simulink model "Inverterfullbridge_rl_load"  (R2023b)
settings: Solver=VariableStepAuto  StartTime=0.0  StopTime=1  RelTol=1e-3
libraries: spsIGBTDiodeLib x4, spsVoltageMeasurementLib x2, spsCurrentMeasurementLib x1, spsDCVoltageSourceLib x1, spsSeriesRLCBranchLib x1, sps_lib x1
settings Model: Creator=junio  LastModifiedBy=Anuj

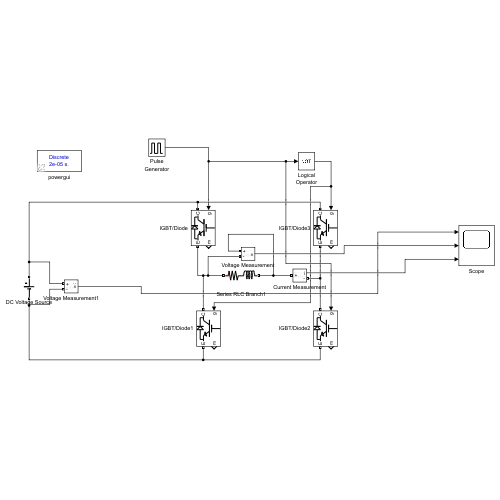
[thumbnail: Simulink's stored preview of the top-level diagram]
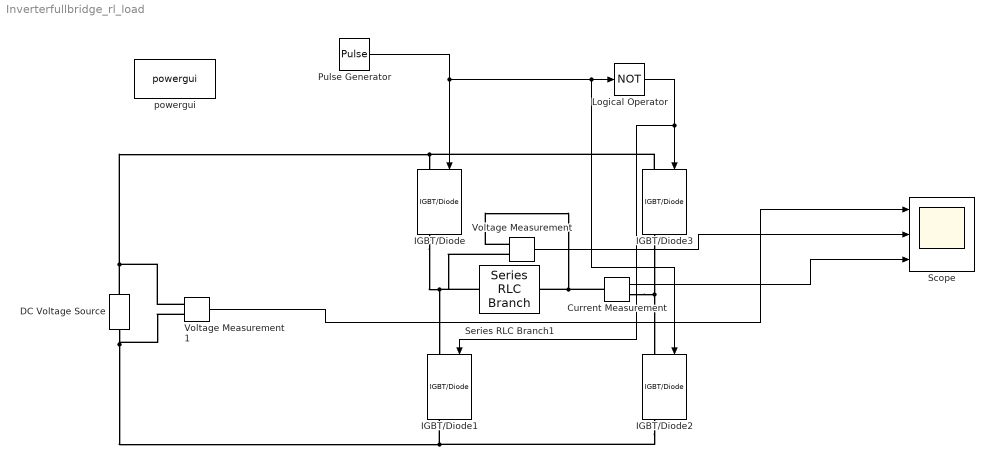
== system Inverterfullbridge_rl_load ==
  Current Measurement : spsCurrentMeasurementLib/Current Measurement  PhasorSimulation=off  OutputType=Complex  PSBequivalent=0
  DC Voltage Source : spsDCVoltageSourceLib/DC Voltage Source  Amplitude=24  Measurements=None
  IGBT/Diode{,1..3} (4 alike) : spsIGBTDiodeLib/IGBT//Diode  Ron=1e-3  Rs=1e5  Cs=inf  Measurements=on
  Logical Operator : Logic  Operator=NOT  AllPortsSameDT=off  OutDataTypeStr=boolean
  Pulse Generator : DiscretePulseGenerator  PulseType=Time based  Period=1/50  PulseWidth=50
  Scope : Scope  NumInputPorts=3
  Series RLC Branch1 : spsSeriesRLCBranchLib/Series RLC Branch  LConnTagsString=__new0  RConnTagsString=__new0  BranchType=RL  Resistance=10  Inductance=5e-3  SetiL0=off  InitialCurrent=0  Capacitance=1e-6  Setx0=off  InitialVoltage=0  Measurements=None
  Voltage Measurement : spsVoltageMeasurementLib/Voltage Measurement  PhasorSimulation=off  OutputType=Complex  PSBequivalent=0
  Voltage Measurement1 : spsVoltageMeasurementLib/Voltage Measurement  PhasorSimulation=off  OutputType=Complex  PSBequivalent=0
  powergui : sps_lib/powergui  Priority=1  SimulationMode=Discrete  SampleTime=2e-05  frequency=60  Iterations=50  frequencyindice=0  Pbase=100e6  ErrMax=1e-4  UnitsV=kV  UnitsW=MW  buscounter=0  FunctionMessages=off  echomessages=off  EnableUseOfTLC=off  CurrentSourceSwitches=off  DisableSnubberDevices=off  DisableRonSwitches=off  DisableVfSwitches=off  DisplayEquations=off  AutomaticDiscreteSolvers=off  SolverType=Tustin/Backward Euler (TBE)  Interpol=off  ExternalGateDelay=off  methode=off  Ts=100  x0status=blocks  SPID=on  SwTol=0  HookPort=off  NonlinearTolerance=1e-4  nMaxIteration=100  ContinueOnMaxIteration=off  RestoreLinks=warning  ResistiveCurrentMeasurement=off  Frange=[0:2:500]  Ylog=off  Xlog=on  ShowGrid=off  save=off  variable=ZData  structure=0  ZoomFFT=off  StartTime=0.0  cycles=1  DisplayStyle=1  fundamental=60  FreqAxis=off  MaxFrequency=1000  frequencyindicesteady=1  RmsSteady=1  display=off
  wires:
  Pulse Generator/1 -> IGBT/Diode2/1, Logical Operator/1, IGBT/Diode/1
  Logical Operator/1 -> IGBT/Diode1/1, IGBT/Diode3/1
  Voltage Measurement1/1 -> Scope/1
  Current Measurement/1 -> Scope/3
  Voltage Measurement/1 -> Scope/2
  connections:
  IGBT/Diode/RConn1 -- Voltage Measurement/LConn2 -- Series RLC Branch1/LConn1 -- IGBT/Diode1/LConn1
  IGBT/Diode3/RConn1 -- Current Measurement/RConn1 -- IGBT/Diode2/LConn1
  DC Voltage Source/RConn1 -- IGBT/Diode3/LConn1 -- IGBT/Diode/LConn1 -- Voltage Measurement1/LConn1
  DC Voltage Source/LConn1 -- IGBT/Diode2/RConn1 -- IGBT/Diode1/RConn1 -- Voltage Measurement1/LConn2
  Current Measurement/LConn1 -- Voltage Measurement/LConn1 -- Series RLC Branch1/RConn1
